simulink model "Exp_8_FWR_2024a"  (R2024a)
settings: Solver=VariableStepAuto  StartTime=0.0  StopTime=0.08  RelTol=1e-3
libraries: fl_lib x10, nesl_utility x3, eeRmsMeasurement x2
settings ModelReferenceCC: UpdateModelReferenceTargets=IfOutOfDate
settings ConfigComp: CovBoundaryAbsTol=1.0e-5
settings SimscapeCC: SimscapeNominalValues="[{\"value\":\"1\",\"unit\":\"A\"},{\"value\":\"1\",\"unit\":\"bar\"},{\"value\":\"1\",\"unit\":\"cm^2\"},{\"value\":\"1\",\"unit\":\"cm^3/s\"},{\"value\":\"1\",\"unit\":\"kJ/kg\"},{\"value\":\"1\",\"unit\":\"kW\"},{\"value\":\"1\",\"unit\":\"l\"},{\"value\":\"1\",\"unit\":\"N\"},{\"value\":\"1\",\"unit\":\"N*m\"},{\"value\":\"1\",\"unit\":\"V\"},{\"value\":\"0.001\",\"unit\":\"Wb\"}]"  SimscapeLogType=all  SimscapeLogDataHistory=10000

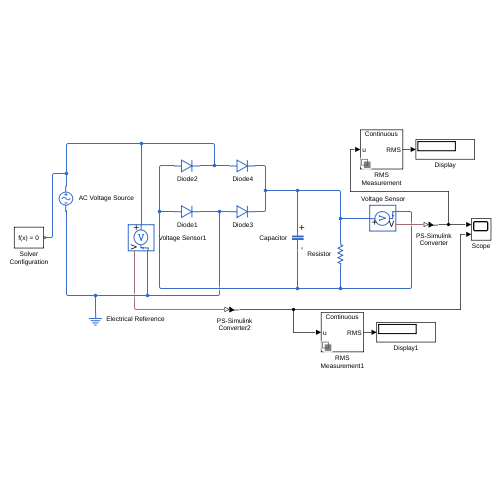
[thumbnail: Simulink's stored preview of the top-level diagram]
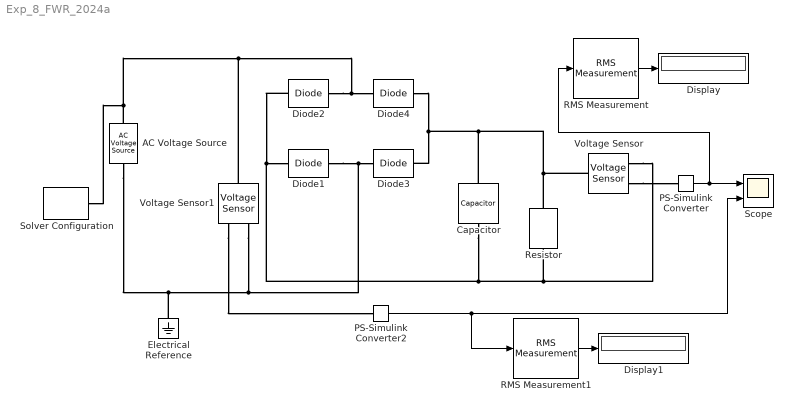
== system Exp_8_FWR_2024a ==
  AC Voltage Source : fl_lib/Electrical/Electrical Sources/AC Voltage Source  amp=5 V  shift=0 deg  frequency=50 Hz
  Capacitor : fl_lib/Electrical/Electrical Elements/Capacitor  c=4700e-6 F  r=1e-6 Ohm  g=0 1/Ohm  i_specify=off  i_priority=None  i=0 A  i_nominal_specify=off  i_nominal_value=1  i_nominal_unit=A  v_specify=off  v_priority=None  v=0 V  v_nominal_specify=off  v_nominal_value=1  v_nominal_unit=V  vc_specify=off  vc_priority=High  vc=0 V  vc_nominal_specify=off  vc_nominal_value=1  vc_nominal_unit=V
  Diode{1..4} (4 alike) : fl_lib/Electrical/Electrical Elements/Diode  Vf=0.7 V  Ron=0.3 Ohm  Goff=1e-8 1/Ohm  i_specify=off  i_priority=None  i=0 A  i_nominal_specify=off  i_nominal_value=1  i_nominal_unit=A  v_specify=off  v_priority=None  v=0 V  v_nominal_specify=off  v_nominal_value=1  v_nominal_unit=V
  Display : Display
  Display1 : Display
  Electrical Reference : fl_lib/Electrical/Electrical Elements/Electrical Reference
  PS-Simulink Converter : nesl_utility/PS-Simulink Converter  PhysicalDomain=network_engine_domain  SubClassName=ps_output  LeftPortType=input  RightPortType=output  PseudoPeriodic=off  Frequencies=[]  VectorFormat=inherit  Unit=inherit  AffineConversion=off
  PS-Simulink Converter2 : nesl_utility/PS-Simulink Converter  PhysicalDomain=network_engine_domain  SubClassName=ps_output  LeftPortType=input  RightPortType=output  PseudoPeriodic=off  Frequencies=[]  VectorFormat=inherit  Unit=inherit  AffineConversion=off
  RMS Measurement : eeRmsMeasurement/RMS Measurement  LabelModeActiveChoice=Total  F=60  SpecifyHarmonics=off  K=[0 1 2]  Ts=0
      settings: LibrarySourceBlock=|
      | ee_sl_lib/Measurements/RMS
      | Measurement
  RMS Measurement1 : eeRmsMeasurement/RMS Measurement  LabelModeActiveChoice=Total  F=60  SpecifyHarmonics=off  K=[0 1 2]  Ts=0
      settings: LibrarySourceBlock=|
      | ee_sl_lib/Measurements/RMS
      | Measurement
  Resistor : fl_lib/Electrical/Electrical Elements/Resistor  R=1 Ohm  i_specify=off  i_priority=None  i=0 A  i_nominal_specify=off  i_nominal_value=1  i_nominal_unit=A  v_specify=off  v_priority=None  v=0 V  v_nominal_specify=off  v_nominal_value=1  v_nominal_unit=V
  Scope : Scope  NumInputPorts=2
  Solver Configuration : nesl_utility/Solver Configuration  PhysicalDomain=network_engine_domain  SubClassName=solver  LeftPortType=input  RightPortType=generic  Tones=[]  Harmonics=[]  SimulateNoise=off  Profile=off  UseLocalSampling=off  EnableSwitchedLinearOptims=on  FrequencyDomain=off  UseCCode=off  RelTol=0.001  AbsTol=0.001  MinStep=1e-09  ToWorkspace=off  RevertToSquareIcSolve=off  NumHomotopyIterations=100  PhasorMode=off  PhasorModeNumHarmonics=1  ConsistencySolver=NEWTON_XTOL_AFTER_FTOL  CanonicalOrdering=CANONICAL  OptimizeIntermediates=OPTIMIZED  IndexReductionMethod=DerivativeReplacement  DoDC=off  ResidualTolerance=1e-09  ConsistencyTolSource=GLOBAL  ConsistencyAbsTol=0.001  ConsistencyRelTol=0.001  ConsistencyTolFactor=0.001  UseLocalSolver=off  LocalSolverChoice=NE_BACKWARD_EULER_ADVANCER  ResolveIndetEquations=on  FunctionEvalNumThread=1  LocalSolverSampleTime=0.001  DoFixedCost=off  MaxNonlinIter=3  MaxModeIter=2  ComputeImpulses=off  ImpulseIterations=2  LinearAlgebra=auto  LinearAlgebraNumThread=0  EquationFormulation=NE_TIME_EF  DelaysMemoryBudget=1024  AutomaticFiltering=on  FilteringTimeConstant=0.001  PartitionStorageMethod=AS_NEEDED  PartitionMemoryBudget=1024  PartitionMethod=ROBUST  MultibodyUseLocalSolver=off  MultibodyLocalSolverChoice=ODE1  MultibodyLocalSolverSampleTime=0.001
  Voltage Sensor : fl_lib/Electrical/Electrical Sensors/Voltage Sensor
  Voltage Sensor1 : fl_lib/Electrical/Electrical Sensors/Voltage Sensor
  wires:
  PS-Simulink Converter/1 -> RMS Measurement/1, Scope/1
  PS-Simulink Converter2/1 -> RMS Measurement1/1, Scope/2
  RMS Measurement/1 -> Display/1
  RMS Measurement1/1 -> Display1/1
  connections:
  Voltage Sensor/RConn1 -- PS-Simulink Converter/LConn1
  Diode2/RConn1 -- Solver Configuration/RConn1 -- AC Voltage Source/LConn1 -- Voltage Sensor1/LConn1 -- Diode4/LConn1
  Diode1/RConn1 -- Electrical Reference/LConn1 -- AC Voltage Source/RConn1 -- Voltage Sensor1/RConn2 -- Diode3/LConn1
  Resistor/RConn1 -- Capacitor/RConn1 -- Diode2/LConn1 -- Diode1/LConn1 -- Voltage Sensor/RConn2
  Diode4/RConn1 -- Capacitor/LConn1 -- Voltage Sensor/LConn1 -- Resistor/LConn1 -- Diode3/RConn1
  Voltage Sensor1/RConn1 -- PS-Simulink Converter2/LConn1
